simulink model "quad_quaternion_tracking_updated"  (R2025b)
settings: Solver=VariableStepAuto  StartTime=0.0  StopTime=59.0  RelTol=1e-3
StopFcn:
  | qsl_post
values from neighbouring files (symbols this model uses):
  g = 9.81    [init_params.m]    (also in init_params_updated.m; qsl_blk_pos.m = cfg.g; qsl_blk_sensors.m = cfg.g)
  J = [Jx Jy Jz]    [init_params.m]    (also in init_params_updated.m)
  m = 0.025    [init_params.m]    (also in init_params_updated.m; qsl_blk_pos.m = cfg.m; qsl_scene.m = 1.5)
  omega0 = [0;0;0]    [init_params.m]    (also in init_params_updated.m)
  q0_init = [1;0;0;0]    [init_params.m]    (also in init_params_updated.m)
  q3r_des = 0    [init_params.m]    (also in init_params_updated.m)
  xi0 = [1.8; 2.27; 0.6]    [init_params.m]    (also in init_params_updated.m)
  xidot0 = [0;0;0]    [init_params.m]    (also in init_params_updated.m)
settings Model: Creator=ASUS  LastModifiedBy=ASUS

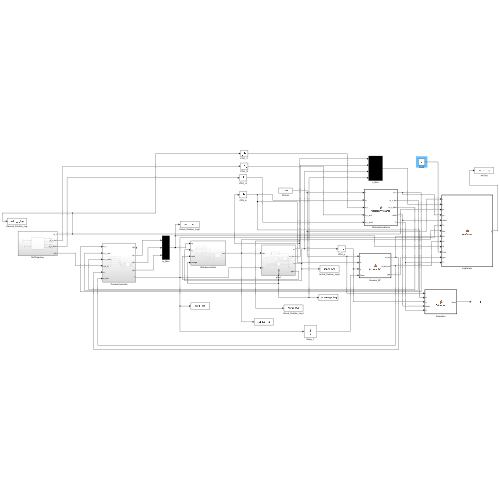
[thumbnail: Simulink's stored preview of the top-level diagram]
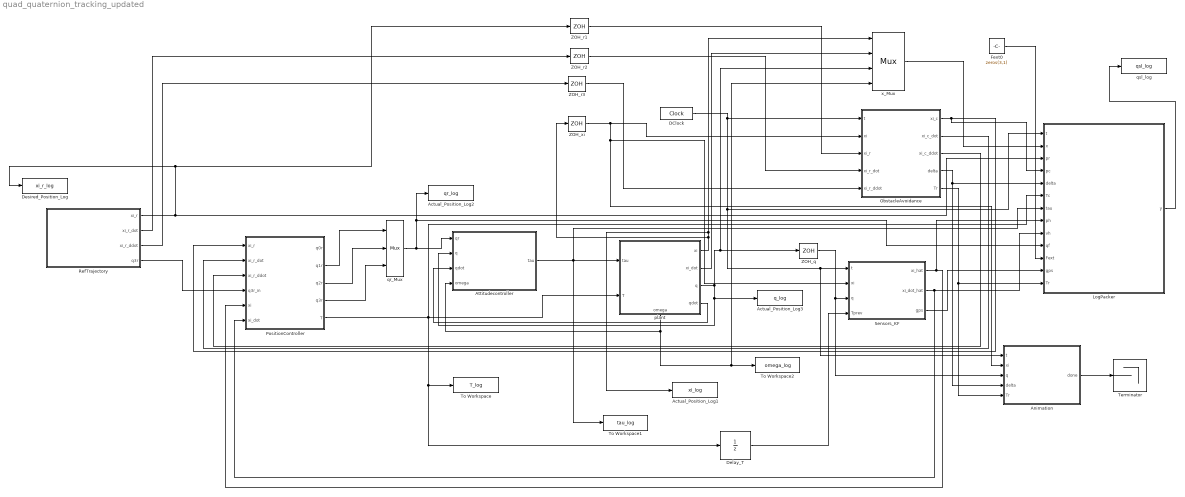
== system quad_quaternion_tracking_updated ==
  Actual_Position_Log1 : ToWorkspace  VariableName=xi_log  SaveFormat=Timeseries  SampleTime=-1
  Actual_Position_Log2 : ToWorkspace  VariableName=qr_log  SaveFormat=Timeseries  SampleTime=-1
  Actual_Position_Log3 : ToWorkspace  VariableName=q_log  SaveFormat=Timeseries  SampleTime=-1
  Animation : MATLAB Function  TreatAsAtomicUnit=on
  Attitudecontroller : Subsystem
  DClock : DigitalClock  SampleTime=0.005
  Delay_T : UnitDelay  InitialCondition=0.025*9.81  SampleTime=0.005  HasFrameUpgradeWarning=on
  Desired_Position_Log : ToWorkspace  VariableName=xi_r_log  SaveFormat=Timeseries  SampleTime=-1
  Fext0 : Constant  Value=zeros(3,1)
  LogPacker : MATLAB Function  TreatAsAtomicUnit=on
  ObstacleAvoidance : MATLAB Function  TreatAsAtomicUnit=on
  PositionController : Subsystem
  RefTrajectory : Subsystem
  Sensors_KF : MATLAB Function  TreatAsAtomicUnit=on
  Terminator : Terminator
  To Workspace : ToWorkspace  VariableName=T_log  SaveFormat=Timeseries  SampleTime=-1
  To Workspace1 : ToWorkspace  VariableName=tau_log  SaveFormat=Timeseries  SampleTime=-1
  To Workspace2 : ToWorkspace  VariableName=omega_log  SaveFormat=Timeseries  SampleTime=-1
  ZOH_q : ZeroOrderHold  SampleTime=-1
  ZOH_r1 : ZeroOrderHold  SampleTime=0.005
  ZOH_r2 : ZeroOrderHold  SampleTime=0.005
  ZOH_r3 : ZeroOrderHold  SampleTime=0.005
  ZOH_xi : ZeroOrderHold  SampleTime=-1
  plant : Subsystem
      settings: PortSchema="{\"entries\":[{\"content\":{\"sides\":[{\"content\":{\"connectorIds\":[\"In1\",\"In2\"]},\"type\":\"ConnectorPlacement.EquallySpacedRectSide\",\"uuid\":\"daf98077-7c24-429b-ae6f-25788d622914\"},{\"content\":{\"connectorIds\":[\"Out1\",\"Out2\",\"Out3\",\"Out4\"],\"side\":\"RIGHT\"},\"type\":\"ConnectorPlacement.EquallySpacedRectSide\",\"uuid\":\"3fd00f15-8adb-4cea-8a6f-ff5caff419f1\"},{\"content\":{\"side\":\"TOP\"},\"type\":\"ConnectorPlacement.EquallySpacedRectSide\",\"uuid\":\"bc39026f-8ae5-435d-80aa-ac75e1f966dc\"},{\"content\":{\"connectorIds\":[\"Out5\"],\"side\":\"BOTTOM\"},\"type\":\"ConnectorPlacement.EquallySpacedRectSide\",\"uuid\":\"f2d81a6b-272d-405c-bcc2-73243a95cee4\"}]},\"type\":\"ConnectorPlacement.EquallySpacedConnector\",\"uuid\":\"f47e6c5f-8c09-48f0-90bc-b2c9317e6b42\"}],\"packageUris\":[\"http://schema.mathworks.com/mf0/Connector/R2020b\"],\"version\":\"1.0\"}"
  qr_Mux : Mux  Inputs=3
  qsl_log : ToWorkspace  VariableName=qsl_log  SampleTime=-1
  x_Mux : Mux
  wires:
  RefTrajectory/1(xi_r) -> LogPacker/3(pr), ZOH_r1/1, Desired_Position_Log/1
  RefTrajectory/2(xi_r_dot) -> ZOH_r2/1
  RefTrajectory/3(xi_r_ddot) -> ZOH_r3/1
  RefTrajectory/4(q3r) -> PositionController/4(q3r_in)
  PositionController/2(q1r) -> qr_Mux/1
  PositionController/3(q2r) -> qr_Mux/2
  PositionController/4(q3r) -> qr_Mux/3
  qr_Mux/1 -> Actual_Position_Log2/1, LogPacker/10(qf), Attitudecontroller/1(qr)
  plant/4(qdot) -> Attitudecontroller/3(qdot)
  plant/5(omega) -> Attitudecontroller/4(omega), x_Mux/4, To Workspace2/1
  Attitudecontroller/1(tau) -> To Workspace1/1, plant/1(tau), LogPacker/7(tau)
  PositionController/5(T) -> To Workspace/1, Delay_T/1, plant/2(T), LogPacker/6(Tc)
  plant/1(xi) -> Actual_Position_Log1/1, x_Mux/1, ZOH_xi/1
  plant/3(q) -> x_Mux/3, ZOH_q/1, Actual_Position_Log3/1, Attitudecontroller/2(q)
  ZOH_r1/1 -> ObstacleAvoidance/3(xi_r)
  ZOH_r2/1 -> ObstacleAvoidance/4(xi_r_dot)
  ZOH_r3/1 -> ObstacleAvoidance/5(xi_r_ddot)
  DClock/1 -> LogPacker/1(t), Animation/1(t), Sensors_KF/1(t), ObstacleAvoidance/1(t)
  ZOH_q/1 -> Sensors_KF/3(q), Animation/3(q)
  ObstacleAvoidance/1(xi_c) -> LogPacker/4(pc), PositionController/1(xi_r)
  ObstacleAvoidance/2(xi_c_dot) -> PositionController/2(xi_r_dot)
  ObstacleAvoidance/3(xi_c_ddot) -> PositionController/3(xi_r_ddot)
  Sensors_KF/1(xi_hat) -> LogPacker/8(ph), PositionController/5(xi)
  Sensors_KF/2(xi_dot_hat) -> LogPacker/9(vh), PositionController/6(xi_dot)
  Delay_T/1 -> Sensors_KF/4(Tprev)
  ZOH_xi/1 -> Animation/2(xi), Sensors_KF/2(xi), ObstacleAvoidance/2(xi)
  ObstacleAvoidance/4(delta) -> LogPacker/5(delta), Animation/4(delta)
  ObstacleAvoidance/5(Tr) -> LogPacker/13(Tr), Animation/5(Tr)
  x_Mux/1 -> LogPacker/2(x)
  Fext0/1 -> LogPacker/11(Fext)
  Sensors_KF/3(gps) -> LogPacker/12(gps)
  LogPacker/1(y) -> qsl_log/1
  plant/2(xi_dot) -> x_Mux/2
  Animation/1(done) -> Terminator/1

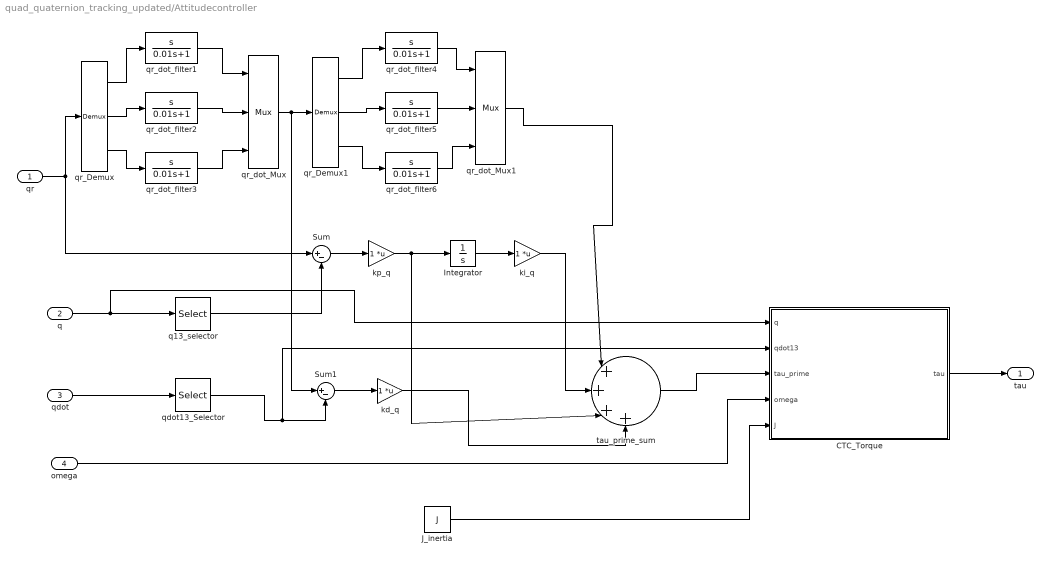
== system quad_quaternion_tracking_updated/Attitudecontroller ==
  qr : Inport
  q : Inport  Port=2
  qdot : Inport  Port=3
  omega : Inport  Port=4
  CTC_Torque : MATLAB Function  TreatAsAtomicUnit=on
  Integrator : Integrator
  J_inertia : Constant  Value=J
  Sum : Sum  Inputs=|+-
  Sum1 : Sum  Inputs=|+-
  kd_q : Gain  Multiplication=Matrix(K*u)
  ki_q : Gain  Multiplication=Matrix(K*u)
  "kp_q " : Gain  Multiplication=Matrix(K*u)
  q13_selector : Selector  InputPortWidth=4  IndexOptions=Index vector (dialog)  Indices=[2:4]  OutputSizes=1
  qdot13_Selector : Selector  InputPortWidth=4  IndexOptions=Index vector (dialog)  Indices=[2:4]  OutputSizes=1
  qr_Demux : Demux  Outputs=3
  qr_Demux1 : Demux  Outputs=3
  qr_dot_Mux : Mux  Inputs=3
  qr_dot_Mux1 : Mux  Inputs=3
  qr_dot_filter{1..6} (6 alike) : TransferFcn  Numerator=[1 0]  Denominator=[0.01 1]
  tau_prime_sum : Sum  Inputs=|++++
  tau : Outport  VectorParamsAs1DForOutWhenUnconnected=off
  wires:
  qr/1 -> qr_Demux/1, Sum/1
  q/1 -> CTC_Torque/1(q), q13_selector/1
  Sum/1 -> "kp_q "/1
  q13_selector/1 -> Sum/2
  Integrator/1 -> ki_q/1
  qdot/1 -> qdot13_Selector/1
  qdot13_Selector/1 -> CTC_Torque/2(qdot13), Sum1/2
  Sum1/1 -> kd_q/1
  qr_dot_Mux1/1 -> tau_prime_sum/1
  ki_q/1 -> tau_prime_sum/2
  "kp_q "/1 -> tau_prime_sum/3, Integrator/1
  kd_q/1 -> tau_prime_sum/4
  tau_prime_sum/1 -> CTC_Torque/3(tau_prime)
  omega/1 -> CTC_Torque/4(omega)
  J_inertia/1 -> CTC_Torque/5(J)
  CTC_Torque/1(tau) -> tau/1
  qr_Demux/1 -> qr_dot_filter1/1
  qr_Demux/2 -> qr_dot_filter2/1
  qr_Demux/3 -> qr_dot_filter3/1
  qr_dot_filter1/1 -> qr_dot_Mux/1
  qr_dot_filter2/1 -> qr_dot_Mux/2
  qr_dot_filter3/1 -> qr_dot_Mux/3
  qr_dot_Mux/1 -> Sum1/1, qr_Demux1/1
  qr_Demux1/1 -> qr_dot_filter4/1
  qr_Demux1/2 -> qr_dot_filter5/1
  qr_Demux1/3 -> qr_dot_filter6/1
  qr_dot_filter4/1 -> qr_dot_Mux1/1
  qr_dot_filter5/1 -> qr_dot_Mux1/2
  qr_dot_filter6/1 -> qr_dot_Mux1/3

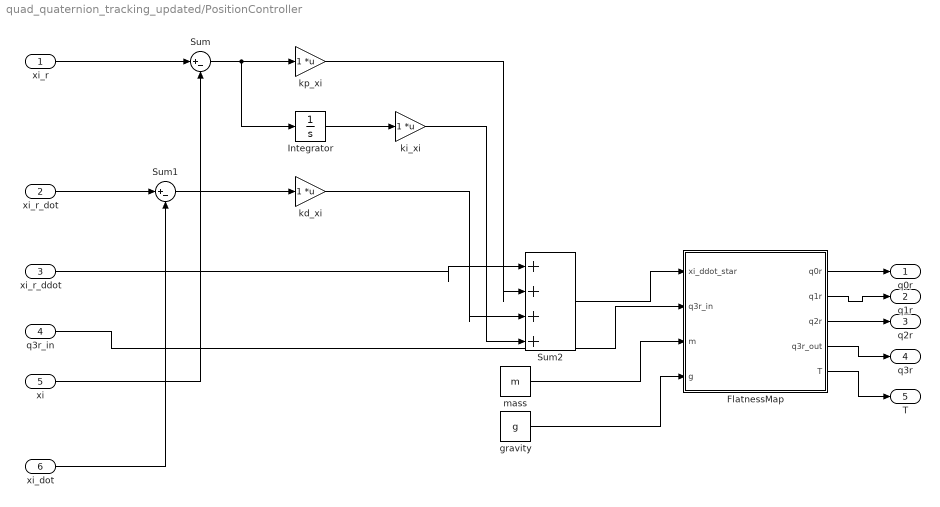
== system quad_quaternion_tracking_updated/PositionController ==
  xi_r : Inport
  xi_r_dot : Inport  Port=2
  xi_r_ddot : Inport  Port=3
  q3r_in : Inport  Port=4
  xi : Inport  Port=5
  xi_dot : Inport  Port=6
  FlatnessMap : MATLAB Function  TreatAsAtomicUnit=on
  Integrator : Integrator
  Sum : Sum  Inputs=|+-
  Sum1 : Sum  Inputs=|+-
  Sum2 : Sum  Inputs=|++++
  gravity : Constant  Value=g
  kd_xi : Gain  Multiplication=Matrix(K*u)
  "ki_xi " : Gain  Multiplication=Matrix(K*u)
  kp_xi : Gain  Multiplication=Matrix(K*u)
  mass : Constant  Value=m
  q0r : Outport  VectorParamsAs1DForOutWhenUnconnected=off
  q1r : Outport  Port=2  VectorParamsAs1DForOutWhenUnconnected=off
  q2r : Outport  Port=3  VectorParamsAs1DForOutWhenUnconnected=off
  q3r : Outport  Port=4  VectorParamsAs1DForOutWhenUnconnected=off
  T : Outport  Port=5  VectorParamsAs1DForOutWhenUnconnected=off
  wires:
  xi_r/1 -> Sum/1
  xi/1 -> Sum/2
  Integrator/1 -> "ki_xi "/1
  kp_xi/1 -> Sum2/2
  xi_r_dot/1 -> Sum1/1
  xi_dot/1 -> Sum1/2
  Sum1/1 -> kd_xi/1
  xi_r_ddot/1 -> Sum2/1
  kd_xi/1 -> Sum2/3
  Sum/1 -> Integrator/1, kp_xi/1
  "ki_xi "/1 -> Sum2/4
  Sum2/1 -> FlatnessMap/1(xi_ddot_star)
  q3r_in/1 -> FlatnessMap/2(q3r_in)
  mass/1 -> FlatnessMap/3(m)
  gravity/1 -> FlatnessMap/4(g)
  FlatnessMap/1(q0r) -> q0r/1
  FlatnessMap/2(q1r) -> q1r/1
  FlatnessMap/3(q2r) -> q2r/1
  FlatnessMap/4(q3r_out) -> q3r/1
  FlatnessMap/5(T) -> T/1

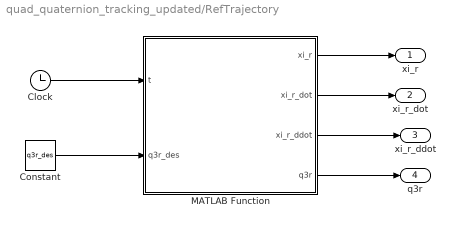
== system quad_quaternion_tracking_updated/RefTrajectory ==
  Clock : Clock
      settings: Decimation=30
  Constant : Constant  Value=q3r_des
  MATLAB Function : MATLAB Function  TreatAsAtomicUnit=on
  xi_r : Outport  VectorParamsAs1DForOutWhenUnconnected=off
  xi_r_dot : Outport  Port=2  VectorParamsAs1DForOutWhenUnconnected=off
  xi_r_ddot : Outport  Port=3  VectorParamsAs1DForOutWhenUnconnected=off
  q3r : Outport  Port=4  VectorParamsAs1DForOutWhenUnconnected=off
  wires:
  Clock/1 -> MATLAB Function/1(t)
  MATLAB Function/1(xi_r) -> xi_r/1
  MATLAB Function/2(xi_r_dot) -> xi_r_dot/1
  MATLAB Function/3(xi_r_ddot) -> xi_r_ddot/1
  MATLAB Function/4(q3r) -> q3r/1
  Constant/1 -> MATLAB Function/2(q3r_des)

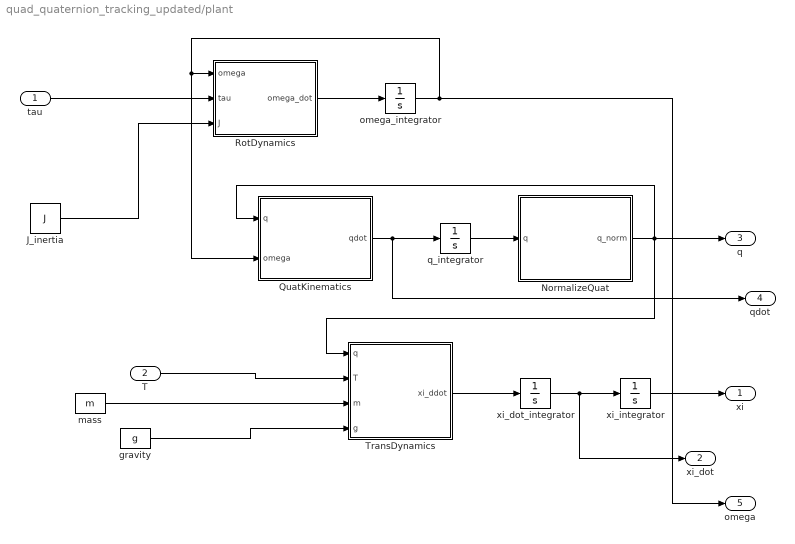
== system quad_quaternion_tracking_updated/plant ==
  tau : Inport
  T : Inport  Port=2
  J_inertia : Constant  Value=J
  NormalizeQuat : MATLAB Function  TreatAsAtomicUnit=on
  QuatKinematics : MATLAB Function  TreatAsAtomicUnit=on
  RotDynamics : MATLAB Function  TreatAsAtomicUnit=on
  TransDynamics : MATLAB Function  TreatAsAtomicUnit=on
  gravity : Constant  Value=g
  mass : Constant  Value=m
  omega_integrator : Integrator  InitialCondition=omega0
  q_integrator : Integrator  InitialCondition=q0_init
  xi_dot_integrator : Integrator  InitialCondition=xidot0
  xi_integrator : Integrator  InitialCondition=xi0
  xi : Outport  VectorParamsAs1DForOutWhenUnconnected=off
  xi_dot : Outport  Port=2  VectorParamsAs1DForOutWhenUnconnected=off
  q : Outport  Port=3  VectorParamsAs1DForOutWhenUnconnected=off
  qdot : Outport  Port=4  VectorParamsAs1DForOutWhenUnconnected=off
  omega : Outport  Port=5  VectorParamsAs1DForOutWhenUnconnected=off
  wires:
  tau/1 -> RotDynamics/2(tau)
  J_inertia/1 -> RotDynamics/3(J)
  RotDynamics/1(omega_dot) -> omega_integrator/1
  omega_integrator/1 -> omega/1, QuatKinematics/2(omega), RotDynamics/1(omega)
  QuatKinematics/1(qdot) -> qdot/1, q_integrator/1
  q_integrator/1 -> NormalizeQuat/1(q)
  NormalizeQuat/1(q_norm) -> TransDynamics/1(q), q/1, QuatKinematics/1(q)
  T/1 -> TransDynamics/2(T)
  mass/1 -> TransDynamics/3(m)
  gravity/1 -> TransDynamics/4(g)
  TransDynamics/1(xi_ddot) -> xi_dot_integrator/1
  xi_dot_integrator/1 -> xi_dot/1, xi_integrator/1
  xi_integrator/1 -> xi/1

== matlab function quad_quaternion_tracking_updated/Sensors_KF ==
  data: t input; xi_hat output; xi input; q input; Tprev input; xi_dot_hat output; gps output
function [xi_hat,xi_dot_hat,gps] = Sensors_KF(t,xi,q,Tprev)
coder.extrinsic('qsl_blk_sensors_exist');
xi_hat=zeros(3,1); xi_dot_hat=zeros(3,1); gps=zeros(3,1);
[xi_hat,xi_dot_hat,gps] = qsl_blk_sensors_exist(t,xi,q,Tprev);

== matlab function quad_quaternion_tracking_updated/Animation ==
  data: t input; done output; xi input; q input; delta input; Tr input
function done = Animation(t,xi,q,delta,Tr)
coder.extrinsic('qsl_blk_anim_exist');
done = 0;
done = qsl_blk_anim_exist(t,xi,q,delta,Tr);

== matlab function quad_quaternion_tracking_updated/LogPacker ==
  data: t input; y output; x input; pr input; pc input; delta input; Tc input; tau input; ph input; vh input; qf input; Fext input; gps input; Tr input
function y = LogPacker(t,x,pr,pc,delta,Tc,tau,ph,vh,qf,Fext,gps,Tr)
     y = [t; x(:); pr(:); pc(:); delta(:); Tc; tau(:); ph(:); vh(:); qf(:); Fext(:); gps(:); Tr(:)];

== matlab function quad_quaternion_tracking_updated/RefTrajectory/MATLAB Function ==
  settings: updateMethod=DISCRETE
  data: t input; xi_r output; xi_r_dot output; xi_r_ddot output; q3r output; q3r_des input
function [xi_r, xi_r_dot, xi_r_ddot, q3r] = RefTrajectoryBSpline(t, q3r_des)
coder.extrinsic('qsl_blk_ref');
xi_r = zeros(3,1); xi_r_dot = zeros(3,1); xi_r_ddot = zeros(3,1);
[xi_r, xi_r_dot, xi_r_ddot] = qsl_blk_ref(t);
q3r = q3r_des;

== matlab function quad_quaternion_tracking_updated/PositionController/FlatnessMap ==
  data: xi_ddot_star input; q0r output; q3r_in input; m input; g input; q1r output; q2r output; q3r_out output; T output
function [q0r,q1r,q2r,q3r_out,T] = FlatnessMap(xi_ddot_star,q3r_in,m,g)

xdd = xi_ddot_star(1);
ydd = xi_ddot_star(2);
zdd = xi_ddot_star(3);

normA = sqrt(xdd^2 + ydd^2 + (zdd+g)^2);

T = m*normA;

q3r_out = q3r_in;

inner = (zdd+g)/normA - 2*q3r_in^2 + 1;

inner = max(inner,0);

sq = sqrt(inner);

q0r = (1/sqrt(2))*sq;

denom = (zdd+g) + normA;

denom = sign(denom)*max(abs(denom),1e-6);

q1r = (xdd*q3r_in - (1/sqrt(2))*ydd*sq)/denom;

q2r = (ydd*q3r_in + (1/sqrt(2))*xdd*sq)/denom;

end

== matlab function quad_quaternion_tracking_updated/Attitudecontroller/CTC_Torque ==
  data: q input; tau output; qdot13 input; tau_prime input; omega input; J input
function tau = CTC_Torque(q, qdot13, tau_prime, omega, J)

Jx = J(1);
Jy = J(2);
Jz = J(3);

Jmat = diag(J);

q0 = q(1);
q1 = q(2);
q2 = q(3);
q3 = q(4);

Q = 2*[ q0  q1  q2  q3;
       -q1  q0  q3 -q2;
       -q2 -q3  q0  q1;
       -q3  q2 -q1  q0];

q0dot = -(q1*qdot13(1) + ...
          q2*qdot13(2) + ...
          q3*qdot13(3)) / max(q0,1e-6);

qdot_full = [q0dot;
             qdot13];

Qq = Q(2:4,:);

tau = Jmat*(Qq*[0;tau_prime]) ...
      + cross(omega,Jmat*omega);

end

== matlab function quad_quaternion_tracking_updated/plant/RotDynamics ==
  data: omega input; omega_dot output; tau input; J input
function omega_dot = RotDynamics(omega,tau,J)

Jx = J(1);
Jy = J(2);
Jz = J(3);

wx = omega(1);
wy = omega(2);
wz = omega(3);

omega_dot = [
    (Jy-Jz)/Jx*wy*wz + tau(1)/Jx;
    (Jz-Jx)/Jy*wz*wx + tau(2)/Jy;
    (Jx-Jy)/Jz*wx*wy + tau(3)/Jz
];

end

== matlab function quad_quaternion_tracking_updated/plant/QuatKinematics ==
  data: q input; qdot output; omega input
function qdot = QuatKinematics(q,omega)

q0 = q(1);
q1 = q(2);
q2 = q(3);
q3 = q(4);

wx = omega(1);
wy = omega(2);
wz = omega(3);

Omega = [
    0  -wx  -wy  -wz;
    wx  0    wz  -wy;
    wy -wz   0    wx;
    wz  wy  -wx   0
];

qdot = 0.5*Omega*q;

end

== matlab function quad_quaternion_tracking_updated/plant/NormalizeQuat ==
  data: q input; q_norm output
function q_norm = NormalizeQuat(q)

q_norm = q / norm(q);

end

== matlab function quad_quaternion_tracking_updated/plant/TransDynamics ==
  data: q input; xi_ddot output; T input; m input; g input
function xi_ddot = TransDynamics(q,T,m,g)

q0 = q(1);
q1 = q(2);
q2 = q(3);
q3 = q(4);

R = [1-2*(q2^2+q3^2),   2*(q1*q2-q0*q3),   2*(q0*q2+q1*q3);
     2*(q1*q2+q0*q3),   1-2*(q1^2+q3^2),   2*(q2*q3-q0*q1);
     2*(q1*q3-q0*q2),   2*(q0*q1+q2*q3),   1-2*(q1^2+q2^2)];

xi_ddot = [0;0;-g] + (T/m)*(R*[0;0;1]);

end

== matlab function quad_quaternion_tracking_updated/ObstacleAvoidance ==
  data: t input; xi_c output; xi input; xi_r input; xi_r_dot input; xi_r_ddot input; xi_c_dot output; xi_c_ddot output; delta output; Tr output
function [xi_c,xi_c_dot,xi_c_ddot,delta,Tr] = ObstacleAvoidance(t,xi,xi_r,xi_r_dot,xi_r_ddot)
coder.extrinsic('qsl_blk_guidance');
xi_c=zeros(3,1); xi_c_dot=zeros(3,1); xi_c_ddot=zeros(3,1); delta=zeros(3,1); Tr=zeros(11,5);
[xi_c,xi_c_dot,xi_c_ddot,delta,Tr] = qsl_blk_guidance(t,xi,xi_r,xi_r_dot,xi_r_ddot);
